simulink model "AXU5EV_Experiment_R5_Algorithms"  (R2026b)
settings: Solver=VariableStepAuto
libraries: simulink x1
settings Model: Creator=lww  LastModifiedBy=lww

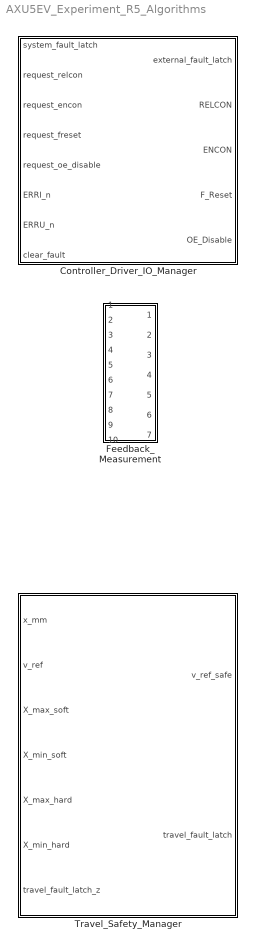
== system AXU5EV_Experiment_R5_Algorithms ==
  Controller_Driver_IO_Manager : Subsystem
  Feedback_Measurement : Subsystem  Description=DSP Caculate_measurement SID465 + count-origin SID1055 and Gain5 SID1058. Reused Delay50/Add1/Gain1. Qualified 100us history, 50 intervals=5ms, 51 observations before valid speed. No IIR. nm_per_count, zero and direction remain explicit inputs. Duplicate frames hold history.
  Travel_Safety_Manager : MATLAB Function  TreatAsAtomicUnit=on

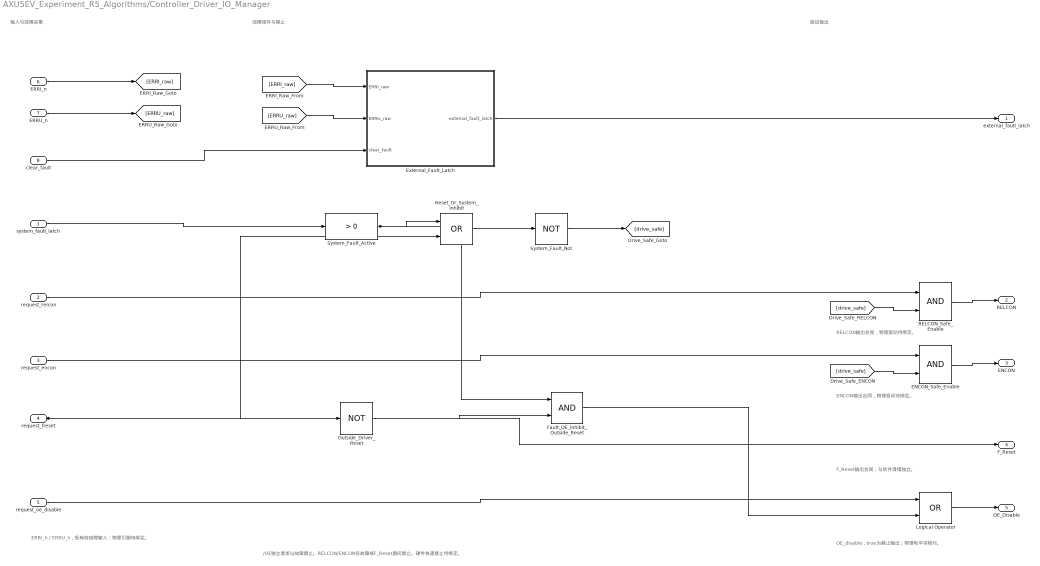
== system AXU5EV_Experiment_R5_Algorithms/Controller_Driver_IO_Manager ==
  note: OE_disable，true为禁止输出；物理电平待核对。
  note: F_Reset输出合同，与软件清错独立。
  note: ENCON输出合同，物理驱动待绑定。
  note: RELCON输出合同，物理驱动待绑定。
  note: ERRI_n / ERRU_n，低有效故障输入；物理引脚待绑定。
  note: /OE独立请求与故障禁止。RELCON/ENCON在故障或F_Reset期间禁止。硬件快速禁止待绑定。
  note: 输入与故障采集
  note: 故障锁存与禁止
  note: 驱动输出
  system_fault_latch : Inport  OutDataTypeStr=boolean  PortDimensions=1
  request_relcon : Inport  Port=2  OutDataTypeStr=boolean  PortDimensions=1  Interpolate=off
  request_encon : Inport  Port=3  OutDataTypeStr=boolean  PortDimensions=1  Interpolate=off
  request_freset : Inport  Port=4  OutDataTypeStr=boolean  PortDimensions=1  Interpolate=off
  request_oe_disable : Inport  Port=5  OutDataTypeStr=boolean  PortDimensions=1  Interpolate=off
  ERRI_n : Inport  Port=6  OutDataTypeStr=boolean  PortDimensions=1  Interpolate=off
  ERRU_n : Inport  Port=7  OutDataTypeStr=boolean  PortDimensions=1  Interpolate=off
  clear_fault : Inport  Port=8  OutDataTypeStr=boolean  PortDimensions=1  Interpolate=off
  ENCON_Safe_Enable : Logic
  External_Fault_Latch : Subsystem
  Fault_OE_Inhibit_Outside_Reset : Logic  AllPortsSameDT=off  OutDataTypeStr=boolean
  Logical Operator : Logic  Operator=OR  AllPortsSameDT=off  OutDataTypeStr=boolean
  Outside_Driver_Reset : Logic  Operator=NOT  Inputs=1  AllPortsSameDT=off  OutDataTypeStr=boolean
  RELCON_Safe_Enable : Logic
  Reset_Or_System_Inhibit : Logic  Operator=OR  AllPortsSameDT=off  OutDataTypeStr=boolean
  System_Fault_Active : simulink/Logic and Bit Operations/Compare To Constant  relop=>  const=0  OutDataTypeStr=boolean
  System_Fault_Not : Logic  Operator=NOT  Inputs=1
  external_fault_latch : Outport  OutDataTypeStr=boolean  PortDimensions=1
  RELCON : Outport  Port=2  OutDataTypeStr=boolean  PortDimensions=1
  ENCON : Outport  Port=3  OutDataTypeStr=boolean  PortDimensions=1
  F_Reset : Outport  Port=4  OutDataTypeStr=boolean  PortDimensions=1
  OE_Disable : Outport  Port=5  OutDataTypeStr=boolean  PortDimensions=1
  wires:
  System_Fault_Not/1 -> [drive_safe]
  request_encon/1 -> ENCON_Safe_Enable/1
  [drive_safe] -> ENCON_Safe_Enable/2
  ERRI_n/1 -> [ERRI_raw]
  ERRU_n/1 -> [ERRU_raw]
  [ERRI_raw] -> External_Fault_Latch/1(ERRI_raw)
  [ERRU_raw] -> External_Fault_Latch/2(ERRU_raw)
  clear_fault/1 -> External_Fault_Latch/3(clear_fault)
  System_Fault_Active/1 -> Fault_OE_Inhibit_Outside_Reset/1, Reset_Or_System_Inhibit/1
  Outside_Driver_Reset/1 -> Fault_OE_Inhibit_Outside_Reset/2
  request_oe_disable/1 -> Logical Operator/1
  Fault_OE_Inhibit_Outside_Reset/1 -> Logical Operator/2
  request_freset/1 -> Outside_Driver_Reset/1, Reset_Or_System_Inhibit/2, F_Reset/1
  request_relcon/1 -> RELCON_Safe_Enable/1
  [drive_safe] -> RELCON_Safe_Enable/2
  system_fault_latch/1 -> System_Fault_Active/1
  Reset_Or_System_Inhibit/1 -> System_Fault_Not/1
  External_Fault_Latch/1(external_fault_latch) -> external_fault_latch/1
  RELCON_Safe_Enable/1 -> RELCON/1
  ENCON_Safe_Enable/1 -> ENCON/1
  Logical Operator/1 -> OE_Disable/1

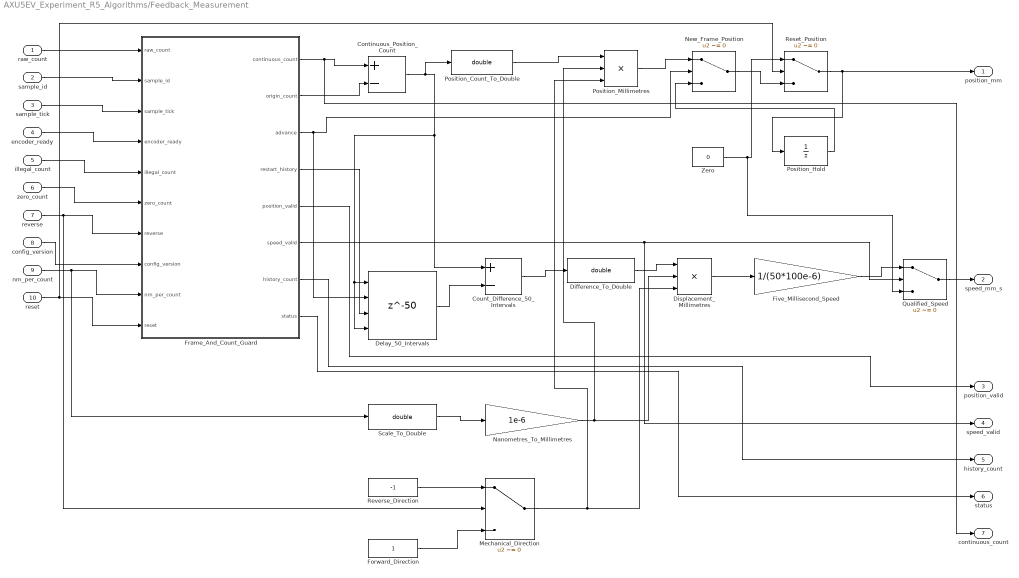
== system AXU5EV_Experiment_R5_Algorithms/Feedback_Measurement ==
  raw_count : Inport  OutDataTypeStr=uint32
  sample_id : Inport  Port=2  OutDataTypeStr=uint32
  sample_tick : Inport  Port=3  OutDataTypeStr=uint64
  encoder_ready : Inport  Port=4  OutDataTypeStr=boolean
  illegal_count : Inport  Port=5  OutDataTypeStr=uint32
  zero_count : Inport  Port=6  OutDataTypeStr=uint32
  reverse : Inport  Port=7  OutDataTypeStr=boolean
  config_version : Inport  Port=8  OutDataTypeStr=uint32
  nm_per_count : Inport  Port=9  OutDataTypeStr=uint32
  reset : Inport  Port=10  OutDataTypeStr=boolean
  Continuous_Position_Count : Sum  Inputs=+-  OutDataTypeStr=int64  AccumDataTypeStr=int64
  Count_Difference_50_Intervals : Sum  Inputs=+-  OutDataTypeStr=int64  AccumDataTypeStr=int64
  Delay_50_Intervals : Delay  DelayLength=50  InitialConditionSource=Input port  ExternalReset=Level hold  ShowEnablePort=on
      settings: InputPortMap=u0,e6,r5,p4
  Difference_To_Double : DataTypeConversion  OutDataTypeStr=double  SaturateOnIntegerOverflow=off  RndMeth=Floor
  Displacement_Millimetres : Product  Inputs=***  OutDataTypeStr=double
  Five_Millisecond_Speed : Gain  Gain=1/(50*100e-6)  OutDataTypeStr=double
  Forward_Direction : Constant  OutDataTypeStr=double
  Frame_And_Count_Guard : MATLAB Function  TreatAsAtomicUnit=on
  Mechanical_Direction : Switch  Criteria=u2 ~= 0  SaturateOnIntegerOverflow=off  InputSameDT=off
  Nanometres_To_Millimetres : Gain  Gain=1e-6  OutDataTypeStr=double
  New_Frame_Position : Switch  Criteria=u2 ~= 0  SaturateOnIntegerOverflow=off  InputSameDT=off
  Position_Count_To_Double : DataTypeConversion  OutDataTypeStr=double  SaturateOnIntegerOverflow=off  RndMeth=Floor
  Position_Hold : UnitDelay  SampleTime=-1
  Position_Millimetres : Product  Inputs=***  OutDataTypeStr=double
  Qualified_Speed : Switch  Criteria=u2 ~= 0  SaturateOnIntegerOverflow=off  InputSameDT=off
  Reset_Position : Switch  Criteria=u2 ~= 0  SaturateOnIntegerOverflow=off  InputSameDT=off
  Reverse_Direction : Constant  Value=-1  OutDataTypeStr=double
  Scale_To_Double : DataTypeConversion  OutDataTypeStr=double  SaturateOnIntegerOverflow=off  RndMeth=Floor
  Zero : Constant  Value=0  OutDataTypeStr=double
  position_mm : Outport  OutDataTypeStr=double
  speed_mm_s : Outport  Port=2  OutDataTypeStr=double
  position_valid : Outport  Port=3  OutDataTypeStr=boolean
  speed_valid : Outport  Port=4  OutDataTypeStr=boolean
  history_count : Outport  Port=5  OutDataTypeStr=uint8
  status : Outport  Port=6  OutDataTypeStr=uint32
  continuous_count : Outport  Port=7  OutDataTypeStr=int64
  wires:
  raw_count/1 -> Frame_And_Count_Guard/1(raw_count)
  sample_id/1 -> Frame_And_Count_Guard/2(sample_id)
  sample_tick/1 -> Frame_And_Count_Guard/3(sample_tick)
  encoder_ready/1 -> Frame_And_Count_Guard/4(encoder_ready)
  illegal_count/1 -> Frame_And_Count_Guard/5(illegal_count)
  zero_count/1 -> Frame_And_Count_Guard/6(zero_count)
  reverse/1 -> Mechanical_Direction/2, Frame_And_Count_Guard/7(reverse)
  config_version/1 -> Frame_And_Count_Guard/8(config_version)
  nm_per_count/1 -> Scale_To_Double/1, Frame_And_Count_Guard/9(nm_per_count)
  reset/1 -> Reset_Position/2, Frame_And_Count_Guard/10(reset)
  Frame_And_Count_Guard/1(continuous_count) -> continuous_count/1, Continuous_Position_Count/1
  Frame_And_Count_Guard/2(origin_count) -> Continuous_Position_Count/2
  Continuous_Position_Count/1 -> Position_Count_To_Double/1, Count_Difference_50_Intervals/1, Delay_50_Intervals/4, Delay_50_Intervals/1
  Scale_To_Double/1 -> Nanometres_To_Millimetres/1
  Reverse_Direction/1 -> Mechanical_Direction/1
  Forward_Direction/1 -> Mechanical_Direction/3
  Position_Count_To_Double/1 -> Position_Millimetres/1
  Nanometres_To_Millimetres/1 -> Position_Millimetres/2, Displacement_Millimetres/2
  Mechanical_Direction/1 -> Position_Millimetres/3, Displacement_Millimetres/3
  Position_Millimetres/1 -> New_Frame_Position/1
  Frame_And_Count_Guard/3(advance) -> Delay_50_Intervals/2, New_Frame_Position/2
  Position_Hold/1 -> New_Frame_Position/3
  Zero/1 -> Qualified_Speed/3, Reset_Position/1
  New_Frame_Position/1 -> Reset_Position/3
  Reset_Position/1 -> Position_Hold/1, position_mm/1
  Frame_And_Count_Guard/4(restart_history) -> Delay_50_Intervals/3
  Delay_50_Intervals/1 -> Count_Difference_50_Intervals/2
  Count_Difference_50_Intervals/1 -> Difference_To_Double/1
  Difference_To_Double/1 -> Displacement_Millimetres/1
  Displacement_Millimetres/1 -> Five_Millisecond_Speed/1
  Five_Millisecond_Speed/1 -> Qualified_Speed/1
  Frame_And_Count_Guard/6(speed_valid) -> speed_valid/1, Qualified_Speed/2
  Qualified_Speed/1 -> speed_mm_s/1
  Frame_And_Count_Guard/5(position_valid) -> position_valid/1
  Frame_And_Count_Guard/7(history_count) -> history_count/1
  Frame_And_Count_Guard/8(status) -> status/1

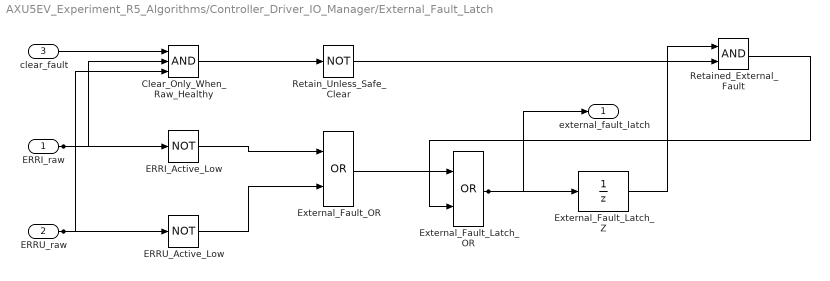
== system AXU5EV_Experiment_R5_Algorithms/Controller_Driver_IO_Manager/External_Fault_Latch ==
  ERRI_raw : Inport  OutDataTypeStr=boolean  PortDimensions=1
  ERRU_raw : Inport  Port=2  OutDataTypeStr=boolean  PortDimensions=1
  clear_fault : Inport  Port=3  OutDataTypeStr=boolean  PortDimensions=1  Interpolate=off
  Clear_Only_When_Raw_Healthy : Logic  Inputs=3  IconShape=distinctive  AllPortsSameDT=off  OutDataTypeStr=boolean
  ERRI_Active_Low : Logic  Operator=NOT  IconShape=distinctive
  ERRU_Active_Low : Logic  Operator=NOT  IconShape=distinctive
  External_Fault_Latch_OR : Logic  Operator=OR  IconShape=distinctive
  External_Fault_Latch_Z : UnitDelay  InitialCondition=false  SampleTime=-1
  External_Fault_OR : Logic  Operator=OR  IconShape=distinctive
  Retain_Unless_Safe_Clear : Logic  Operator=NOT  Inputs=1  IconShape=distinctive  AllPortsSameDT=off  OutDataTypeStr=boolean
  Retained_External_Fault : Logic  IconShape=distinctive  AllPortsSameDT=off  OutDataTypeStr=boolean
  external_fault_latch : Outport  OutDataTypeStr=boolean  PortDimensions=1
  wires:
  Retained_External_Fault/1 -> External_Fault_Latch_OR/2
  Retain_Unless_Safe_Clear/1 -> Retained_External_Fault/2
  External_Fault_Latch_Z/1 -> Retained_External_Fault/1
  Clear_Only_When_Raw_Healthy/1 -> Retain_Unless_Safe_Clear/1
  clear_fault/1 -> Clear_Only_When_Raw_Healthy/1
  External_Fault_Latch_OR/1 -> External_Fault_Latch_Z/1, external_fault_latch/1
  External_Fault_OR/1 -> External_Fault_Latch_OR/1
  ERRU_Active_Low/1 -> External_Fault_OR/2
  ERRI_Active_Low/1 -> External_Fault_OR/1
  ERRU_raw/1 -> Clear_Only_When_Raw_Healthy/3, ERRU_Active_Low/1
  ERRI_raw/1 -> ERRI_Active_Low/1, Clear_Only_When_Raw_Healthy/2

== matlab function AXU5EV_Experiment_R5_Algorithms/Feedback_Measurement/Frame_And_Count_Guard ==
  data: raw_count input; continuous_count output; sample_id input; sample_tick input; encoder_ready input; illegal_count input; zero_count input; reverse input; config_version input; nm_per_count input; reset input; origin_count output; advance output; restart_history output; position_valid output; speed_valid output; history_count output; status output
function [continuous_count,origin_count,advance,restart_history,position_valid,speed_valid,history_count,status] = f(raw_count,sample_id,sample_tick,encoder_ready,illegal_count,zero_count,reverse,config_version,nm_per_count,reset)
%#codegen
[continuous_count,origin_count,advance,restart_history,position_valid,speed_valid,history_count,status]=axu5ev_experiment_encoder_guard(raw_count,sample_id,sample_tick,encoder_ready,illegal_count,zero_count,reverse,config_version,nm_per_count,reset);
end

== matlab function AXU5EV_Experiment_R5_Algorithms/Travel_Safety_Manager ==
  data: v_ref_safe output; x_mm input; travel_fault_latch output; v_ref input; X_max_soft input; X_min_soft input; X_max_hard input; X_min_hard input; travel_fault_latch_z input
function [v_ref_safe, travel_fault_latch] = Travel_Safety_Manager( ...
    x_mm, v_ref, X_max_soft, X_min_soft, X_max_hard, X_min_hard, travel_fault_latch_z)
% PMLSM travel safety manager
% 功能：
% 1. 软限位：只限制继续向越界方向运动，不触发硬关断
% 2. 硬限位：触发 travel_fault_latch，锁存故障
% 3. travel_fault_latch = 1 后，v_ref_safe 强制为 0
% 注意：
% 上一拍锁存由外部状态块保持，明确安全清除输入控制其复位。
% PI_Reset、Init_Reset 与驱动 F_Reset 保持各自职责。
% 速度方向判断死区，单位 mm/s
V_eps = 0.0;

% ---------- 1. 硬限位检测 ----------
hard_hi = (x_mm >= X_max_hard);
hard_lo = (x_mm <= X_min_hard);
hard_fault_raw = hard_hi || hard_lo;

% ---------- 2. 外部锁存 ----------
% 上一拍已经故障，或者当前触发硬限位，则继续保持故障
fault_latch_now = (travel_fault_latch_z > 0.5) || hard_fault_raw;

% ---------- 3. 软限位方向性限制 ----------
right_soft = (x_mm >= X_max_soft);
left_soft  = (x_mm <= X_min_soft);

v_pos_dir = (v_ref >  V_eps);
v_neg_dir = (v_ref < -V_eps);

right_block = right_soft && v_pos_dir;
left_block  = left_soft  && v_neg_dir;

soft_block = right_block || left_block;

% ---------- 4. 输出安全速度 ----------
if fault_latch_now
    v_ref_safe = 0.0;
elseif soft_block
    v_ref_safe = 0.0;
else
    v_ref_safe = v_ref;
end

travel_fault_latch = double(fault_latch_now);
end
